simulink subsystem "Kalman_Filter_sub"  (R2023b)
settings: Solver=VariableStepAuto  StartTime=0.0  StopTime=10.0  RelTol=1e-3
undefined symbols (not defined in the file): Discrete, KF_Enable, KF_Vision_Covariance, t_sample, Time
libraries: simulink x2, ctrlSharedLib x1
settings Model: Creator=ander  LastModifiedBy=ander

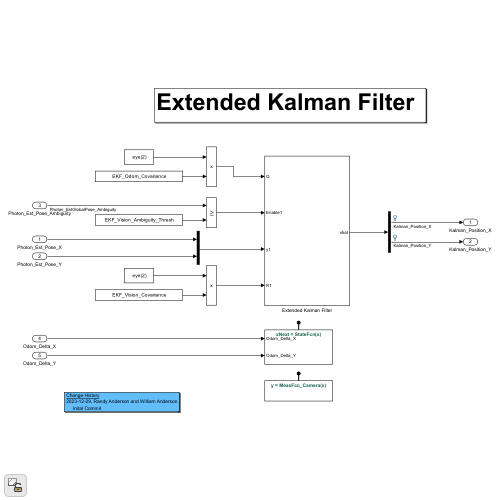
[thumbnail: Simulink's stored preview of the top-level diagram]
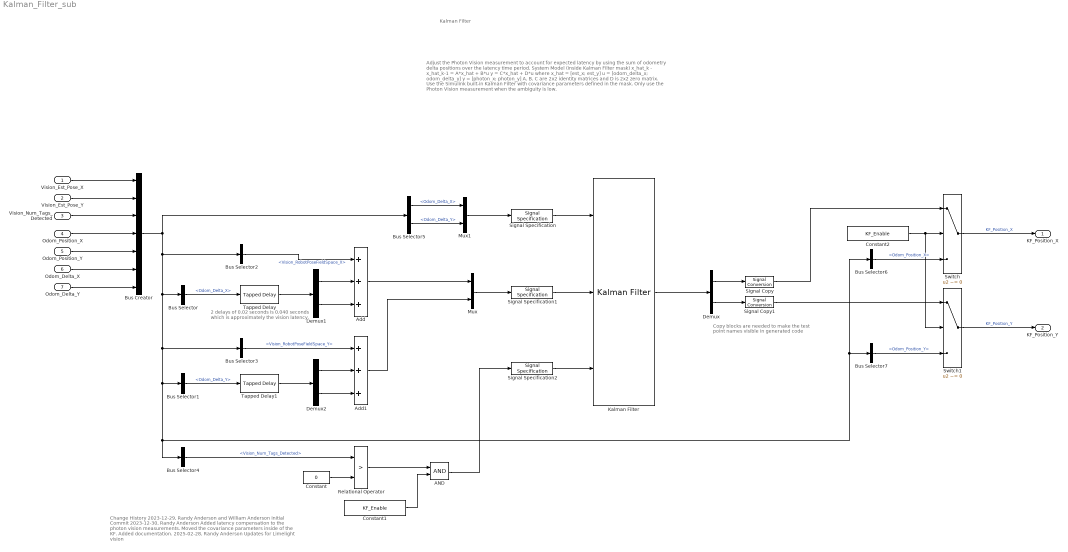
== system Kalman_Filter_sub ==
  note: Adjust the Photon Vision measurement to account for expected latency by using the sum of odometry delta positions over the latency time period.
      |
      | System Model (inside Kalman Filter mask)
      |    x_hat_k - x_hat_k-1 = A*x_hat + B*u
      |    y                               = C*x_hat + D*u
      |
      | where
      |    x_hat = [est_x; est_y]
      |    u = [odom_delta_x; odom_delta_y]
      |    y = [photon_x; photon_y]
      |    A, B, C are 2x2 identity matrices and D is 2x2 zero matrix.
      |
      | Use the Simulink built-in Kalman Filter with covariance parameters defined in the mask.
      |
      | Only use the Photon Vision measurement when the ambiguity is low.
  note: 2 delays of 0.02 seconds is 0.040 seconds which is approximately the vision latency.
  note: Copy blocks are needed to make the test point names visible in generated code
  note: Change History
      | 2023-12-29, Randy Anderson and William Anderson
      | Initial Commit
      | 2023-12-30, Randy Anderson
      | Added latency compensation to the photon vision measurements.
      | Moved the covariance parameters inside of the KF.
      | Added documentation.
      | 2025-02-28, Randy Anderson
      | Updates for Limelight vision
  note: Kalman Filter
  Vision_Est_Pose_X : Inport
  Vision_Est_Pose_Y : Inport  Port=2
  Vision_Num_Tags_Detected : Inport  Port=3
  Odom_Position_X : Inport  Port=4
  Odom_Position_Y : Inport  Port=5
  Odom_Delta_X : Inport  Port=6
  Odom_Delta_Y : Inport  Port=7
  AND : Logic  AllPortsSameDT=off  OutDataTypeStr=boolean
  Add : Sum  Inputs=3
  Add1 : Sum  Inputs=3
  Bus Creator : BusCreator  Inputs=7
  Bus Selector : BusSelector  OutputSignals=Odom_Delta_X
  Bus Selector1 : BusSelector  OutputSignals=Odom_Delta_Y
  Bus Selector2 : BusSelector  OutputSignals=Vision_RobotPoseFieldSpace_X
  Bus Selector3 : BusSelector  OutputSignals=Vision_RobotPoseFieldSpace_Y
  Bus Selector4 : BusSelector  OutputSignals=Vision_Num_Tags_Detected
  Bus Selector5 : BusSelector  OutputSignals=Odom_Delta_X,Odom_Delta_Y
  Bus Selector6 : BusSelector  OutputSignals=Odom_Position_X
  Bus Selector7 : BusSelector  OutputSignals=Odom_Position_Y
  Constant : Constant  Value=0
  Constant1 : Constant  Value=KF_Enable
  Constant2 : Constant  Value=KF_Enable
  Demux : Demux  Outputs=2
  Demux1 : Demux  Outputs=2
  Demux2 : Demux  Outputs=2
  Kalman Filter : ctrlSharedLib/Kalman Filter  TimeDomain=Discrete-Time  UseCurrentEstimator=on  ModelSource=Individual A, B, C, D matrices  ModelSourceVariable=ss(0.95,1,1,0,1)  A=eye(2)  B=eye(2)  C=eye(2)  D=eye(2)*0  NumberOfStates=1  NumberOfInputs=1  NumberOfOutputs=1  InitialEstimateSource=Dialog  X0=[0;0]  P0=10  UseK=off  UseGH=off  NumberOfProcessNoiseInputs=1  G=eye(2)  TimeInvariantG=on  H=eye(2)*1e-2  TimeInvariantH=on  Q=KF_Odom_Covariance  TimeInvariantQ=on  R=KF_Vision_Covariance  TimeInvariantR=on  N=0  TimeInvariantN=on  AddInputPort=on  AddEnablePort=on  OutputEstimatedY=off  OutputP=off  Ts=t_sample
  Mux : Mux  Inputs=2
  Mux1 : Mux  Inputs=2
  Relational Operator : RelationalOperator  Operator=>  OutDataTypeStr=boolean  RndMeth=Simplest  InputSameDT=off
  Signal Copy : SignalConversion  OverrideOpt=off
  Signal Copy1 : SignalConversion  OverrideOpt=off
  Signal Specification : SignalSpecification  SampleTime=t_sample
  Signal Specification1 : SignalSpecification  SampleTime=t_sample
  Signal Specification2 : SignalSpecification  SampleTime=t_sample
  Switch : Switch  Criteria=u2 ~= 0  SaturateOnIntegerOverflow=off  InputSameDT=off
  Switch1 : Switch  Criteria=u2 ~= 0  SaturateOnIntegerOverflow=off  InputSameDT=off
  Tapped Delay : simulink/Discrete/Tapped Delay  vinit=0.0  samptime=-1  NumDelays=2  DelayOrder=Oldest  includeCurrent=off
  Tapped Delay1 : simulink/Discrete/Tapped Delay  vinit=0.0  samptime=-1  NumDelays=2  DelayOrder=Oldest  includeCurrent=off
  KF_Position_X : Outport
  KF_Position_Y : Outport  Port=2
  wires:
  Kalman Filter/1 -> Demux/1
  Mux/1 -> Signal Specification1/1
  Mux1/1 -> Signal Specification/1
  Constant/1 -> Relational Operator/2
  Demux/2 -> Signal Copy1/1
  Demux/1 -> Signal Copy/1
  Signal Specification/1 -> Kalman Filter/1
  Signal Specification1/1 -> Kalman Filter/2
  Signal Specification2/1 -> Kalman Filter/3
  Tapped Delay/1 -> Demux1/1
  Vision_Est_Pose_X/1 -> Bus Creator/1
  Vision_Est_Pose_Y/1 -> Bus Creator/2
  Vision_Num_Tags_Detected/1 -> Bus Creator/3
  Bus Creator/1 -> Bus Selector2/1, Bus Selector/1, Bus Selector3/1, Bus Selector1/1, Bus Selector6/1, Bus Selector7/1, Bus Selector4/1, Bus Selector5/1
  Bus Selector/1 -> Tapped Delay/1  "<Odom_Delta_X>"
  Demux1/1 -> Add/2
  Demux1/2 -> Add/3
  Demux2/2 -> Add1/3
  Demux2/1 -> Add1/2
  Tapped Delay1/1 -> Demux2/1
  Bus Selector1/1 -> Tapped Delay1/1  "<Odom_Delta_Y>"
  Bus Selector3/1 -> Add1/1  "<Vision_RobotPoseFieldSpace_Y>"
  Bus Selector2/1 -> Add/1  "<Vision_RobotPoseFieldSpace_X>"
  Add/1 -> Mux/1
  Add1/1 -> Mux/2
  Bus Selector4/1 -> Relational Operator/1  "<Vision_Num_Tags_Detected>"
  Bus Selector5/1 -> Mux1/1  "<Odom_Delta_X>"
  Bus Selector5/2 -> Mux1/2  "<Odom_Delta_Y>"
  Relational Operator/1 -> AND/1
  AND/1 -> Signal Specification2/1
  Constant1/1 -> AND/2
  Constant2/1 -> Switch/2, Switch1/2
  Switch/1 -> KF_Position_X/1  "KF_Position_X"
  Switch1/1 -> KF_Position_Y/1  "KF_Position_Y"
  Signal Copy/1 -> Switch/1
  Signal Copy1/1 -> Switch1/1
  Odom_Position_X/1 -> Bus Creator/4
  Odom_Position_Y/1 -> Bus Creator/5
  Odom_Delta_X/1 -> Bus Creator/6
  Odom_Delta_Y/1 -> Bus Creator/7
  Bus Selector6/1 -> Switch/3  "<Odom_Position_X>"
  Bus Selector7/1 -> Switch1/3  "<Odom_Position_Y>"
